simulink model "HIamp_record_LSL_DD_vMMR_new"  (R2020a)
settings: Solver=FixedStepDiscrete  StartTime=0.0  StopTime=10000  FixedStep=1/600  RelTol=1e-3
libraries: LSL x1, DataAcquisition x1
settings Model: Creator=AvivaLab  LastModifiedBy=AvivaLab
settings SolverCC: AutoInsertRateTranBlk=on

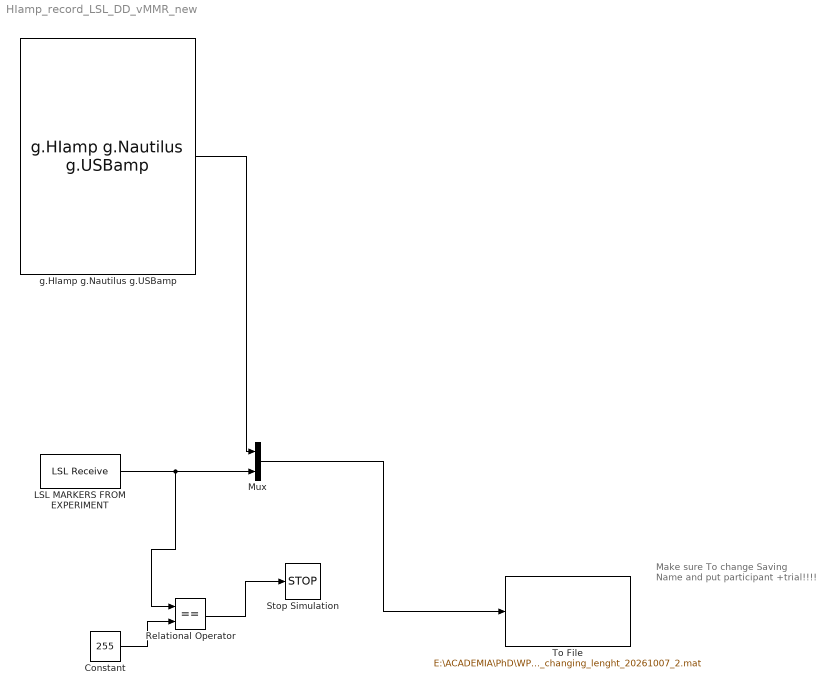
== system HIamp_record_LSL_DD_vMMR_new ==
  note: Make sure To change Saving Name and put participant +trial!!!!
  Constant : Constant  Value=255
  LSL MARKERS FROM EXPERIMENT : LSL/LSL Receive  noChannels=1  lslPropName=name  lslPropValue='experiment_markers'  sampleRate=200
      settings: SourceProductName=g.HIsys
  Mux : Mux  Inputs=2
  Relational Operator : RelationalOperator  Operator===  OutDataTypeStr=boolean  RndMeth=Simplest
  Stop Simulation : Stop
  To File : ToFile  Filename=E:\ACADEMIA\PhD\WP5\EEG_Recordings\Photodiode_Calib_vMMR\photodiode_test_changing_lenght_20261007_2.mat  MatrixName=EEG_data
  g.HIamp g.Nautilus g.USBamp : DataAcquisition/g.HIamp g.Nautilus g.USBamp  cfgUpdated=740262.5856  numDevices=2  deviceSR=[500 250 ]  deviceChannels=[9 4 ]  numSR=[2 ]  SRIndexPerDevice=[1 0 ]
      settings: SourceProductName=g.HIsys
  wires:
  g.HIamp g.Nautilus g.USBamp/1 -> Mux/1
  LSL MARKERS FROM EXPERIMENT/1 -> Relational Operator/1, Mux/2
  Mux/1 -> To File/1
  Relational Operator/1 -> Stop Simulation/1
  Constant/1 -> Relational Operator/2
